simulink model "secorddiagfs"  (R2024a)
settings: Solver=VariableStepAuto  StartTime=0.0  StopTime=2  RelTol=1e-3
libraries: simulink_extras x1, cstblocks x1, dspobslib x1
settings Model: Creator=eniya  LastModifiedBy=SHASHANK DADURIA

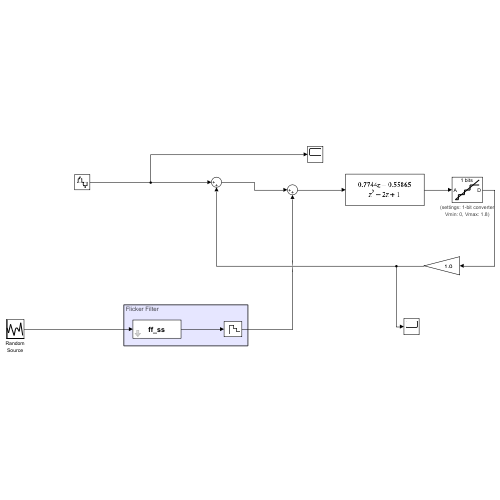
[thumbnail: Simulink's stored preview of the top-level diagram]
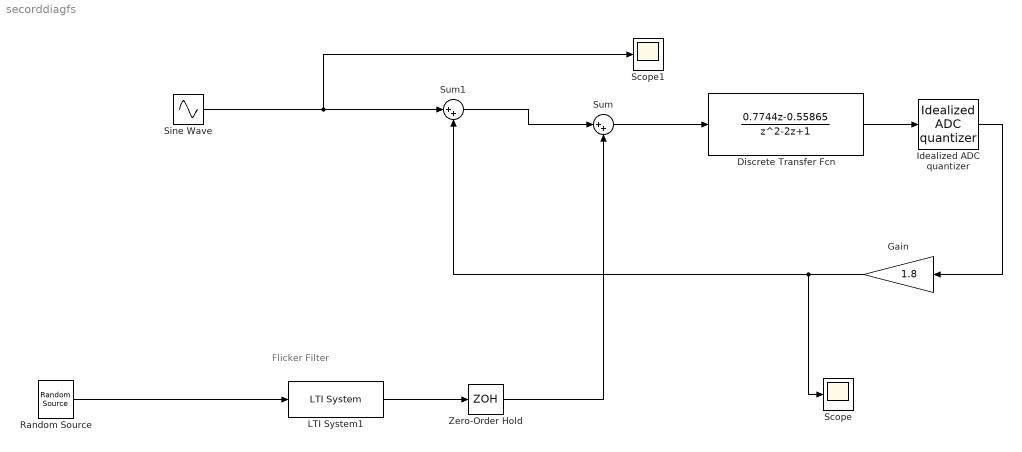
== system secorddiagfs ==
  note: Flicker Filter
  Discrete Transfer Fcn : DiscreteTransferFcn  Numerator="[0.7744  -0.55865]"  Denominator=[1 -2 1]
  Gain : Gain  Gain=1.8
  Idealized ADC quantizer : simulink_extras/Additional Discrete/Idealized ADC quantizer  NumberOfConverterBits=1  Vmin=0  Vmax=1.8  OutputDataType=int32  OutputNegativeValues=off
  LTI System1 : cstblocks/LTI System  sys=ff_ss  IC=[]  PadeOrder=0
  Random Source : dspobslib/Random Source  SrcType=Gaussian  NormMethod=Ziggurat  CltLength=12  MinVal=0  MaxVal=1  MeanVal=0  VarVal=1e-8  RepMode=Not repeatable  rawSeed=1  IsInherit=off  SampMode=Discrete  SampTime=1/(2000*1024)  SampFrame=1  DataType=Double  OutComplex=Real  OutputFrames=off
  Scope : Scope
  Scope1 : Scope
  Sine Wave : Sin  Amplitude=0.65  Bias=0.9  Frequency=((2000*64)*127*32*4*2*pi)/(32768*128)  SampleTime=1/(2000*1024)
  Sum : Sum  Inputs=|++
  Sum1 : Sum  Inputs=|++
  Zero-Order Hold : ZeroOrderHold  SampleTime=1/(2000*1024)
  wires:
  Discrete Transfer Fcn/1 -> Idealized ADC quantizer/1
  Gain/1 -> Sum1/2, Scope/1
  Idealized ADC quantizer/1 -> Gain/1
  Sine Wave/1 -> Sum1/1, Scope1/1
  Sum/1 -> Discrete Transfer Fcn/1
  Sum1/1 -> Sum/1
  Zero-Order Hold/1 -> Sum/2
  Random Source/1 -> LTI System1/1
  LTI System1/1 -> Zero-Order Hold/1
